simulink model "enr312_motor_identified"  (R2026a)
settings: Solver=ode1  StopTime=Tend  FixedStep=dt
model workspace (MAT data in the model file):
  K = 1
  Kd = 0
  Ki = 1.5
  Kp = 0.3
  Tend = 5
  Tf = 0.01
  Ts = 0.1
  aTF = 0.990049833749
  acc = 50
  blWidth = 1e-09
  closedLoop = 1
  dt = 0.001
  dz = 0
  latency = 0.07
  measSel = 1
  qCnt = 1
  qSpd = 4.615
  sensorAtLoad = 0
  spProfile = [0 60]
  theta = 0
  uMax = 180
libraries: slpidlib x1, simulink x1
settings Model: Creator=odyssix  LastModifiedBy=odyssix

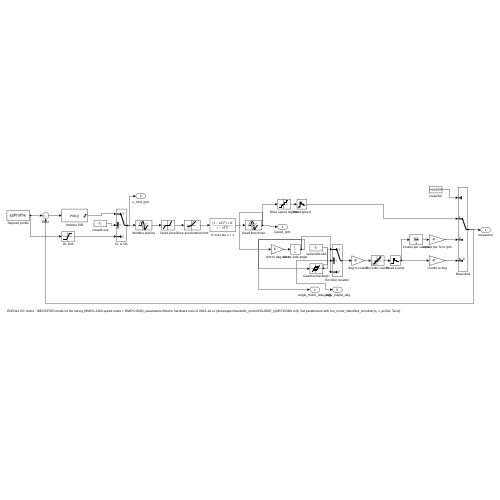
[thumbnail: Simulink's stored preview of the top-level diagram]
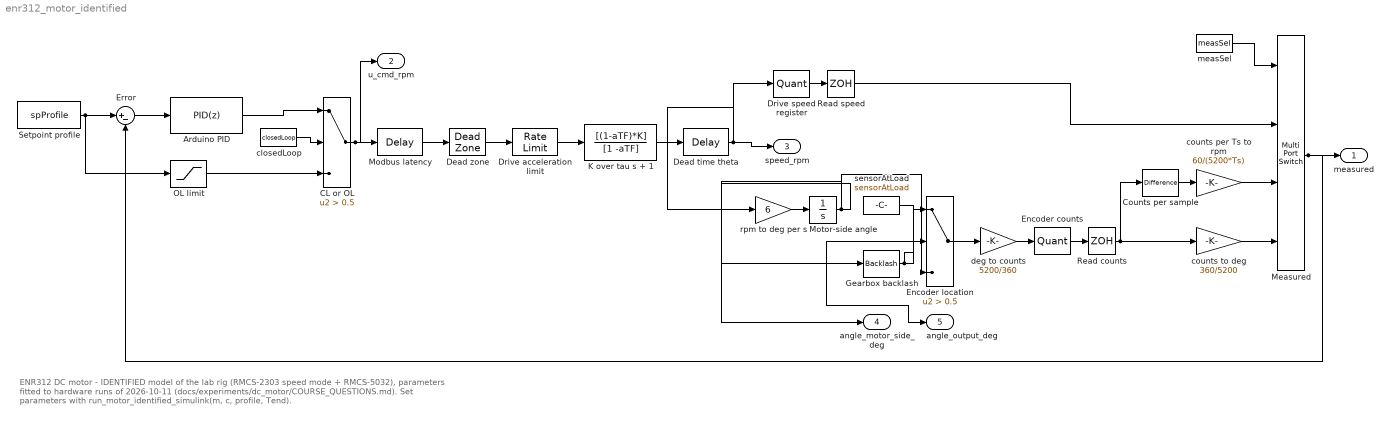
== system enr312_motor_identified ==
  note: ENR312 DC motor - IDENTIFIED model of the lab rig (RMCS-2303 speed mode + RMCS-5032), parameters fitted to hardware runs of 2026-10-11 (docs/experiments/dc_motor/COURSE_QUESTIONS.md). Set parameters with run_motor_identified_simulink(m, c, profile, Tend).
  Arduino PID : slpidlib/PID Controller  Controller=PID  Form=Parallel  TimeDomain=Discrete-time  UseExternalTs=off  SampleTime=Ts  IntegratorMethod=Backward Euler  FilterMethod=Backward Euler  ControllerParametersSource=internal  P=Kp  I=Ki  UseKiTs=off  D=Kd  UseExternalDerivativeSource=off  N=1/Tf  UseFilter=on  TunerSelectOption=Transfer Function Based (PID Tuner App)  InitialConditionSource=internal  InitialConditionForIntegrator=0  InitialConditionForFilter=0  DifferentiatorICPrevScaledInput=0  ExternalReset=none  TrackingMode=off  Kt=1  LimitOutput=on  SatLimitsSource=internal  UpperSaturationLimit=uMax  LowerSaturationLimit=-uMax  LinearizeAsGain=off  AntiWindupMode=clamping  Kb=1  LimitIntegrator=off  UpperIntegratorSaturationLimit=inf  LowerIntegratorSaturationLimit=-inf  POutMin=[]  POutMax=[]  IOutMin=[]  IOutMax=[]  DOutMin=[]  DOutMax=[]  NOutMin=[]  NOutMax=[]  SumOutMin=[]  SumOutMax=[]  SaturationOutMin=[]  SaturationOutMax=[]  PParamMin=[]  PParamMax=[]  IParamMin=[]  IParamMax=[]  DParamMin=[]  DParamMax=[]  NParamMin=[]  NParamMax=[]  KbParamMin=[]  KbParamMax=[]  KtParamMin=[]  KtParamMax=[]  KbOutMin=[]  KbOutMax=[]  KtOutMin=[]  KtOutMax=[]  IntegratorOutMin=[]  IntegratorOutMax=[]  FilterOutMin=[]  FilterOutMax=[]  SumI1OutMin=[]  SumI1OutMax=[]  SumI2OutMin=[]  SumI2OutMax=[]  SumI3OutMin=[]  SumI3OutMax=[]  SumI4OutMin=[]  SumI4OutMax=[]  SumDOutMin=[]  SumDOutMax=[]  DifferentiatorOutMin=[]  DifferentiatorOutMax=[]  FilterDiffOutCoefMin=[]  FilterDiffOutCoefMax=[]  ReciprocalOutMin=[]  ReciprocalOutMax=[]  SumDenOutMin=[]  SumDenOutMax=[]  SumNumOutMin=[]  SumNumOutMax=[]  DivideOutMin=[]  DivideOutMax=[]  UdiffTsProdOutMin=[]  UdiffTsProdOutMax=[]  NTsProdOutMin=[]  NTsProdOutMax=[]  UintegralTsProdOutMin=[]  UintegralTsProdOutMax=[]  UngainTsProdOutMin=[]  UngainTsProdOutMax=[]  ClampingZeroOutDataTypeStr=Inherit: Inherit via back propagation  ClampingZeroOutMin=[]  ClampingZeroOutMax=[]  FilterDenConstantOutDataTypeStr=Inherit: Inherit via back propagation  FilterDenConstantOutMin=[]  FilterDenConstantOutMax=[]  PCopyOutDataTypeStr=Inherit: Inherit via back propagation  PCopyOutMin=[]  PCopyOutMax=[]  NCopyOutDataTypeStr=Inherit: Inherit via back propagation  NCopyOutMin=[]  NCopyOutMax=[]  IntegratorContinuousStateAttributes=''  IntegratorStateMustResolveToSignalObject=off  IntegratorRTWStateStorageClass=Auto  FilterContinuousStateAttributes=''  FilterStateMustResolveToSignalObject=off  FilterRTWStateStorageClass=Auto  ParallelPVariant=InternalParameters  IdealPVariant=Disabled  IVariant=InternalParameters  DVariant=InternalParameters  IntegratorVariant=Discrete  SatVariant=Enabled  AWVariant=DiscClampingParallel  PCopyVariant=Disabled  TRVariant=Disabled  FdbkBlocksVariant=Feedback  IdealPFdbkVariant=Passthrough  SatFdbkVariant=Passthrough  DerivativeFilterVariant=BackwardEulerFilter  NVariant=InternalParameters  NCopyVariant=InternalParameters  FilterICVariant=InternalICsFilter  IntegratorICVariant=InternalICs  ExternalResetVariant=Disabled  TRSumVariant=Passthrough  SumFdbkVariant=Enabled  SumVariant=Sum_PID  TsampFilterVariant=InternalTs  TsampNgainVariant=Passthrough  TsampIntegralVariant=Disabled_SignalSpec  ExternalSaturationOutDataTypeStr=Inherit: Same as second input  DerivativeSourceVariant=ErrorSignal  PreIntVariant=InternalPreInt
      settings: LibrarySourceBlock=simulink/Discrete/Discrete PID Controller
  CL or OL : Switch  Criteria=u2 > Threshold  Threshold=0.5  SaturateOnIntegerOverflow=off  InputSameDT=off
  Counts per sample : simulink/Discrete/Difference  ICPrevInput=0.0  OutMin=[]  OutMax=[]  OutDataType=fixdt(1, 16)  OutScaling=2^-10  DoSatur=off
  Dead time theta : TransportDelay  DelayTime=theta
  Dead zone : DeadZone  LowerValue=-dz  UpperValue=dz
  Drive acceleration limit : RateLimiter  RisingSlewLimit=acc  FallingSlewLimit=-acc  SampleTimeMode=inherited
  Drive speed register : Quantizer  QuantizationInterval=qSpd
  Encoder counts : Quantizer  QuantizationInterval=qCnt
  Encoder location : Switch  Criteria=u2 > Threshold  Threshold=0.5  SaturateOnIntegerOverflow=off  InputSameDT=off
  Error : Sum  Inputs=|+-
  Gearbox backlash : Backlash  BacklashWidth=blWidth
  K over tau s + 1 : DiscreteTransferFcn  Numerator=[(1-aTF)*K]  Denominator=[1 -aTF]  SampleTime=dt
  Measured : MultiPortSwitch  SaturateOnIntegerOverflow=off  InputSameDT=off
  Modbus latency : TransportDelay  DelayTime=latency
  Motor-side angle : Integrator
  OL limit : Saturate  UpperLimit=uMax  LowerLimit=-uMax
  Read counts : ZeroOrderHold  SampleTime=Ts
  Read speed : ZeroOrderHold  SampleTime=Ts
  Setpoint profile : FromWorkspace  VariableName=spProfile  SampleTime=Ts  Interpolate=off  OutputAfterFinalValue=Holding final value
  closedLoop : Constant  Value=closedLoop
  counts per Ts to rpm : Gain  Gain=60/(5200*Ts)
  counts to deg : Gain  Gain=360/5200
  deg to counts : Gain  Gain=5200/360
  measSel : Constant  Value=measSel
  rpm to deg per s : Gain  Gain=6
  sensorAtLoad : Constant  Value=sensorAtLoad
  measured : Outport
  u_cmd_rpm : Outport  Port=2
  speed_rpm : Outport  Port=3
  angle_motor_side_deg : Outport  Port=4
  angle_output_deg : Outport  Port=5
  wires:
  Setpoint profile/1 -> Error/1, OL limit/1
  Error/1 -> Arduino PID/1
  Arduino PID/1 -> CL or OL/1
  closedLoop/1 -> CL or OL/2
  OL limit/1 -> CL or OL/3
  CL or OL/1 -> u_cmd_rpm/1, Modbus latency/1
  Modbus latency/1 -> Dead zone/1
  Dead zone/1 -> Drive acceleration limit/1
  Drive acceleration limit/1 -> K over tau s + 1/1
  K over tau s + 1/1 -> Dead time theta/1
  Dead time theta/1 -> speed_rpm/1, rpm to deg per s/1, Drive speed register/1
  rpm to deg per s/1 -> Motor-side angle/1
  Motor-side angle/1 -> Gearbox backlash/1, angle_motor_side_deg/1, Encoder location/3
  Gearbox backlash/1 -> angle_output_deg/1, Encoder location/1
  Drive speed register/1 -> Read speed/1
  sensorAtLoad/1 -> Encoder location/2
  Encoder location/1 -> deg to counts/1
  deg to counts/1 -> Encoder counts/1
  Encoder counts/1 -> Read counts/1
  Read counts/1 -> Counts per sample/1, counts to deg/1
  Counts per sample/1 -> counts per Ts to rpm/1
  measSel/1 -> Measured/1
  Read speed/1 -> Measured/2
  counts per Ts to rpm/1 -> Measured/3
  counts to deg/1 -> Measured/4
  Measured/1 -> Error/2, measured/1
